simulink model "SDID_test"  (Simulink 4.00)
settings: Solver=ode45  StartTime=0.0  StopTime=2000.0  RelTol=1e-3
libraries: simulink3 x2, libsb2sl x1
settings Model: LastModifiedBy=k079210  LimitDataPoints=off

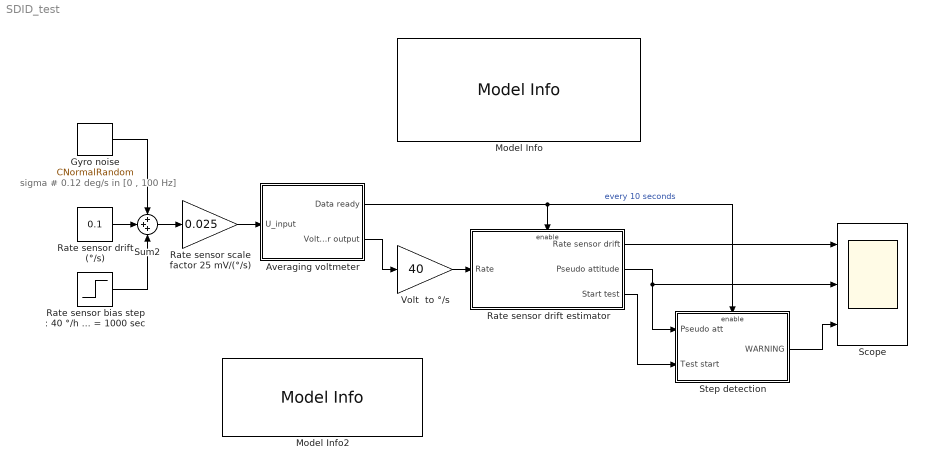
== system SDID_test ==
  note: sigma # 0.12 deg/s
      | in [0 , 100 Hz]
  Averaging voltmeter : Subsystem
      settings: RTWFcnNameOpts=Auto  RTWFileNameOpts=Auto
  Gyro noise : libsb2sl/SNG/CNormalRandom  SEED=7  T0=0  MEAN=0.000000  STD=0.12  INTM=Linear  TS=0.01
  Model Info : simulink3/Signals & Systems/Model Info  InitialBlockCM=None  BlockCM=None  Frame=on  DisplayStringWithTags=|  HorizontalTextAlignment=Center  LeftAlignmentValue=0.5  SourceBlockDiagram=SDID_test  TagMaxNumber=20
      | RATE SENSOR TEST
      | ----------------------------------
      | 
      | 
      | Thales Avionics / JRC
      | October 2002
  Model Info2 : simulink3/Signals & Systems/Model Info  InitialBlockCM=None  BlockCM=None  Frame=on  DisplayStringWithTags=|  HorizontalTextAlignment=Center  LeftAlignmentValue=0.5  SourceBlockDiagram=SDID_test  TagMaxNumber=20
      | This test has to be performed at ambiant
      | room temperature, so that rate sensor
      | output should remain constant.
  "Rate sensor bias step : 40 °/h at t = 1000 sec" : Step  Time=1000  Before=0  After=40/3600  SampleTime=0
  Rate sensor drift (°/s) : Constant  Value=0.1
  Rate sensor drift estimator : Subsystem  TreatAsAtomicUnit=on
      settings: RTWFcnNameOpts=Auto  RTWFileNameOpts=Auto
  Rate sensor scale factor 25 mV/(°/s) : Gain  Gain=0.025  Multiplication=Element-wise(K.*u)  SaturateOnIntegerOverflow=on
  Scope : Scope  NumInputPorts=3
      settings: TimeRange=auto  YMin=0.0975~-1.5~0  YMax=0.115~3~1  SaveToWorkspace=off  SaveName=ScopeData  MaxDataPoints=5000  Decimation=10
  Step detection : Subsystem  TreatAsAtomicUnit=on
      settings: RTWFcnNameOpts=Auto  RTWFileNameOpts=Auto
  Sum2 : Sum  Inputs=+++  SaturateOnIntegerOverflow=on
  Volt  to °/s : Gain  Gain=40  Multiplication=Element-wise(K.*u)  SaturateOnIntegerOverflow=on
  wires:
  Gyro noise/1 -> Sum2/1
  "Rate sensor bias step : 40 °/h at t = 1000 sec"/1 -> Sum2/3
  Averaging voltmeter/1(Data ready) -> Step detection/Enable, Rate sensor drift estimator/Enable  "every 10 seconds"
  Sum2/1 -> Rate sensor scale factor 25 mV/(°/s)/1
  Rate sensor scale factor 25 mV/(°/s)/1 -> Averaging voltmeter/1(U_input)
  Averaging voltmeter/2(Voltmeter output) -> Volt  to °/s/1
  Volt  to °/s/1 -> Rate sensor drift estimator/1(Rate)
  Rate sensor drift (°/s)/1 -> Sum2/2
  Rate sensor drift estimator/1(Rate sensor drift) -> Scope/1
  Rate sensor drift estimator/2(Pseudo attitude) -> Step detection/1(Pseudo att), Scope/2
  Rate sensor drift estimator/3(Start test) -> Step detection/2(Test start)
  Step detection/1(WARNING) -> Scope/3

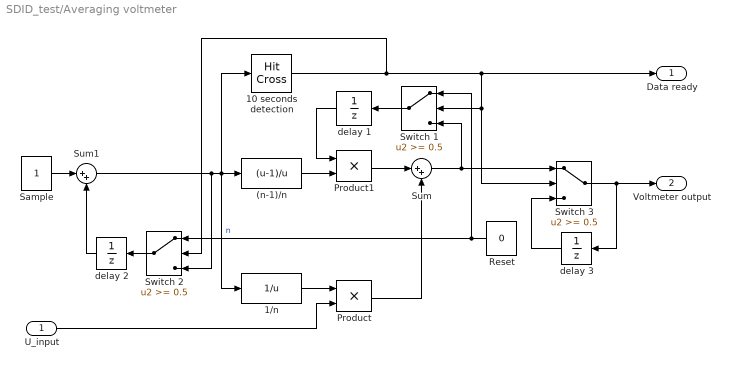
== system SDID_test/Averaging voltmeter ==
  U_input : Inport  Port=1  LatchInput=off
  (n-1)/n : Fcn  Expr=(u-1)/u
  1/n : Fcn  Expr=1/u
  10 seconds detection : HitCross  HitCrossingOffset=1000  HitCrossingDirection=either  ShowOutputPort=on
  Product : Product  Inputs=2  Multiplication=Element-wise(.*)  SaturateOnIntegerOverflow=on
  Product1 : Product  Inputs=2  Multiplication=Element-wise(.*)  SaturateOnIntegerOverflow=on
  Reset : Constant  Orientation=left  Value=0
  Sample : Constant  Value=1
  Sum : Sum  Inputs=|++  SaturateOnIntegerOverflow=on
  Sum1 : Sum  Inputs=|++  SaturateOnIntegerOverflow=on
  Switch 1 : Switch  Orientation=left  Threshold=0.5
  Switch 2 : Switch  Orientation=left  Threshold=0.5
  Switch 3 : Switch  Threshold=0.5
  delay 1 : UnitDelay  Orientation=left  X0=0  SampleTime=0.01
      settings: RTWStateStorageClass=Auto
  delay 2 : UnitDelay  Orientation=left  X0=0  SampleTime=0.01
      settings: RTWStateStorageClass=Auto
  delay 3 : UnitDelay  Orientation=left  X0=0  SampleTime=0.01
      settings: RTWStateStorageClass=Auto
  Data ready : Outport  Port=1
  Voltmeter output : Outport  Port=2
  wires:
  1/n/1 -> Product/1
  Product/1 -> Sum/2
  (n-1)/n/1 -> Product1/2
  Product1/1 -> Sum/1
  Sum/1 -> Switch 1/3, Switch 3/1
  delay 1/1 -> Product1/1
  U_input/1 -> Product/2
  Switch 1/1 -> delay 1/1
  Sample/1 -> Sum1/1
  Sum1/1 -> (n-1)/n/1, 1/n/1, 10 seconds detection/1, Switch 2/3  "n"
  delay 2/1 -> Sum1/2
  Switch 2/1 -> delay 2/1
  10 seconds detection/1 -> Switch 2/2, Switch 1/2, Switch 3/2, Data ready/1
  Reset/1 -> Switch 2/1, Switch 1/1
  delay 3/1 -> Switch 3/3
  Switch 3/1 -> delay 3/1, Voltmeter output/1

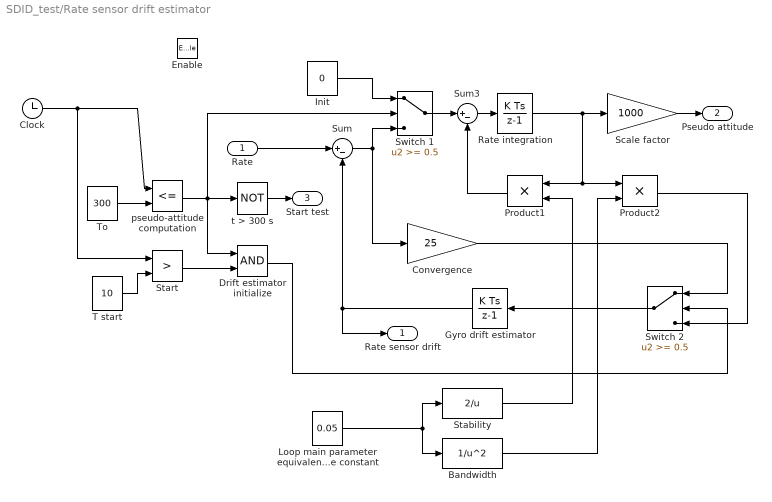
== system SDID_test/Rate sensor drift estimator ==
  Rate : Inport  Port=1  LatchInput=off
  Enable : EnablePort
  Bandwidth : Fcn  Expr=1/u^2
  Clock : Clock
      settings: DisplayTime=off
  Convergence : Gain  Gain=25  Multiplication=Element-wise(K.*u)  SaturateOnIntegerOverflow=on
  Drift estimator initialize : Logic  Operator=AND  Inputs=2
  Gyro drift estimator : DiscreteIntegrator  Orientation=left  IntegratorMethod=ForwardEuler  ExternalReset=none  InitialConditionSource=internal  InitialCondition=0  LimitOutput=off  UpperSaturationLimit=inf  LowerSaturationLimit=-inf  ShowSaturationPort=off  ShowStatePort=off  SampleTime=0.01
      settings: RTWStateStorageClass=Auto
  Init : Constant  Value=0
  Loop main parameter equivalent to time constant : Constant  Value=0.05
  Product1 : Product  Orientation=left  Inputs=2  Multiplication=Element-wise(.*)  SaturateOnIntegerOverflow=on
  Product2 : Product  Inputs=2  Multiplication=Element-wise(.*)  SaturateOnIntegerOverflow=on
  Rate integration : DiscreteIntegrator  IntegratorMethod=ForwardEuler  ExternalReset=none  InitialConditionSource=internal  InitialCondition=0  LimitOutput=off  UpperSaturationLimit=inf  LowerSaturationLimit=-inf  ShowSaturationPort=off  ShowStatePort=off  SampleTime=0.01
      settings: RTWStateStorageClass=Auto
  Scale factor : Gain  Gain=1000  Multiplication=Element-wise(K.*u)  SaturateOnIntegerOverflow=on
  Stability : Fcn  Expr=2/u
  Start : RelationalOperator  Operator=>
  Sum : Sum  Inputs=|+-  SaturateOnIntegerOverflow=on
  Sum3 : Sum  Inputs=|+-  SaturateOnIntegerOverflow=on
  Switch 1 : Switch  Threshold=0.5
  Switch 2 : Switch  Orientation=left  Threshold=0.5
  T start : Constant  Value=10
  To : Constant  Value=300
  pseudo-attitude computation : RelationalOperator  Operator=<=
  t > 300 s : Logic  Operator=NOT  Inputs=2
  Rate sensor drift : Outport  Port=1
  Pseudo attitude : Outport  Port=2
  Start test : Outport  Port=3
  wires:
  pseudo-attitude computation/1 -> Drift estimator initialize/1, Switch 1/2, t > 300 s/1
  Product2/1 -> Switch 2/3
  Product1/1 -> Sum3/2
  Switch 2/1 -> Gyro drift estimator/1
  Drift estimator initialize/1 -> Switch 2/2
  Start/1 -> Drift estimator initialize/2
  T start/1 -> Start/2
  Init/1 -> Switch 1/1
  Sum/1 -> Switch 1/3, Convergence/1
  Switch 1/1 -> Sum3/1
  Sum3/1 -> Rate integration/1
  Rate/1 -> Sum/1
  To/1 -> pseudo-attitude computation/2
  Clock/1 -> pseudo-attitude computation/1, Start/1
  Convergence/1 -> Switch 2/1
  Loop main parameter equivalent to time constant/1 -> Stability/1, Bandwidth/1
  Stability/1 -> Product1/2
  Bandwidth/1 -> Product2/2
  Rate integration/1 -> Product1/1, Product2/1, Scale factor/1
  Gyro drift estimator/1 -> Sum/2, Rate sensor drift/1
  Scale factor/1 -> Pseudo attitude/1
  t > 300 s/1 -> Start test/1

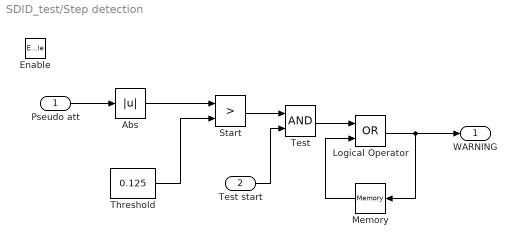
== system SDID_test/Step detection ==
  Pseudo att : Inport  Port=1  LatchInput=off
  Test start : Inport  Port=2  LatchInput=off
  Enable : EnablePort
  Abs : Abs  SaturateOnIntegerOverflow=on
  Logical Operator : Logic  Operator=OR  Inputs=2
  Memory : Memory  Orientation=left  X0=0  InheritSampleTime=off
      settings: RTWStateStorageClass=Auto
  Start : RelationalOperator  Operator=>
  Test : Logic  Operator=AND  Inputs=2
  Threshold : Constant  Value=0.125
  WARNING : Outport  Port=1
  wires:
  Logical Operator/1 -> WARNING/1, Memory/1
  Memory/1 -> Logical Operator/2
  Threshold/1 -> Start/2
  Start/1 -> Test/1
  Test/1 -> Logical Operator/1
  Test start/1 -> Test/2
  Abs/1 -> Start/1
  Pseudo att/1 -> Abs/1
